simulink model "zad31"  (R2022b)
settings: Solver=FixedStepAuto  StartTime=0.0  StopTime=50  FixedStep=0.00001  RelTol=1e-3
model workspace (MAT data in the model file):
  a0 = 1
  a1 = 1
undefined symbols (not defined in the file): Ki, Kp
settings Model: Creator=vandm  LastModifiedBy=vandm

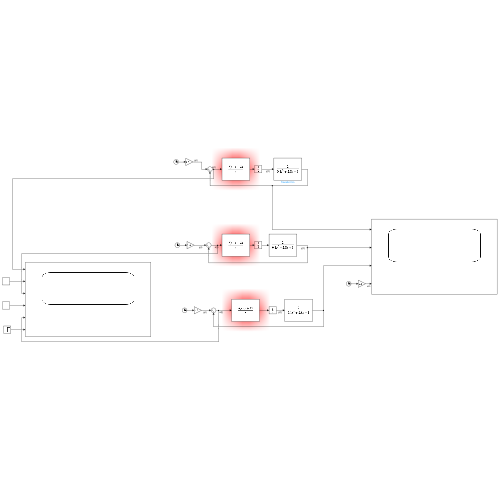
[thumbnail: Simulink's stored preview of the top-level diagram]
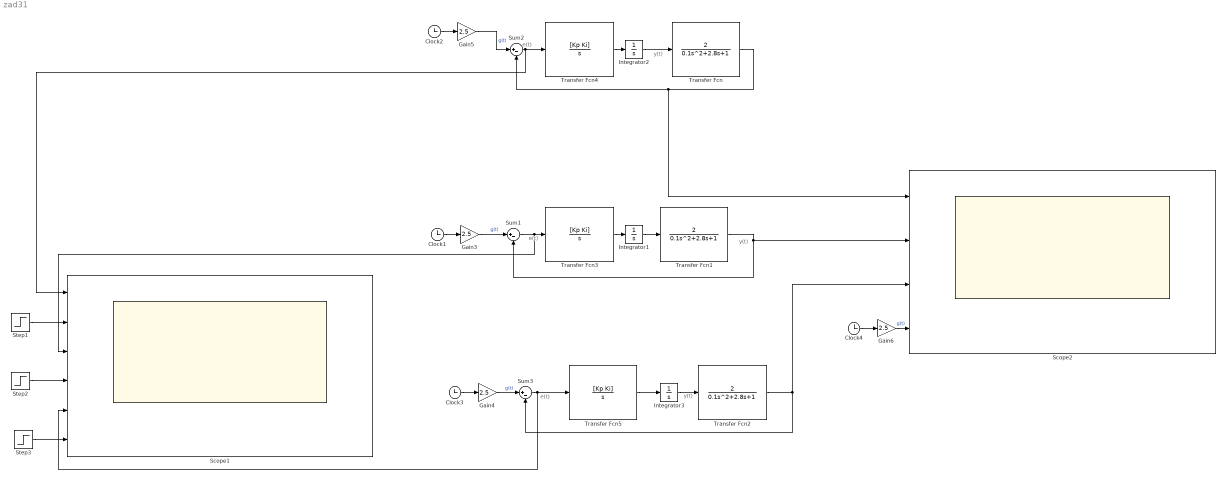
== system zad31 ==
  note: e(t)
  note: y(t)
  note: y(t)
  note: e(t)
  note: y(t)
  note: e(t)
  Clock{1..4} (4 alike) : Clock
  Gain{3..6} (4 alike) : Gain  Gain=2.5
  Integrator1 : Integrator
  Integrator2 : Integrator
  Integrator3 : Integrator
  Scope1 : Scope  NumInputPorts=6
  Scope2 : Scope  NumInputPorts=4
  Step1 : Step  Time=0  After=2.5/(2*1)  SampleTime=0
  Step2 : Step  Time=0  After=2.5/(2*5)  SampleTime=0
  Step3 : Step  Time=0  After=2.5/(2*10)  SampleTime=0
  Sum1 : Sum  Inputs=|+-
  Sum2 : Sum  Inputs=|+-
  Sum3 : Sum  Inputs=|+-
  Transfer Fcn : TransferFcn  Numerator=[2]  Denominator=[0.1 2.8 1]
  Transfer Fcn1 : TransferFcn  Numerator=[2]  Denominator=[0.1 2.8 1]
  Transfer Fcn2 : TransferFcn  Numerator=[2]  Denominator=[0.1 2.8 1]
  Transfer Fcn3 : TransferFcn  Numerator=[Kp Ki]  Denominator=[1 0]
  Transfer Fcn4 : TransferFcn  Numerator=[Kp Ki]  Denominator=[1 0]
  Transfer Fcn5 : TransferFcn  Numerator=[Kp Ki]  Denominator=[1 0]
  wires:
  Gain5/1 -> Sum2/1  "g(t)"
  Sum2/1 -> Transfer Fcn4/1, Scope1/1
  Integrator2/1 -> Transfer Fcn/1
  Transfer Fcn/1 -> Scope2/1, Sum2/2
  Gain3/1 -> Sum1/1  "g(t)"
  Integrator1/1 -> Transfer Fcn1/1
  Transfer Fcn1/1 -> Sum1/2, Scope2/2
  Transfer Fcn2/1 -> Sum3/2, Scope2/3
  Gain4/1 -> Sum3/1  "g(t)"
  Integrator3/1 -> Transfer Fcn2/1
  Sum3/1 -> Transfer Fcn5/1, Scope1/5
  Clock2/1 -> Gain5/1
  Clock1/1 -> Gain3/1
  Clock3/1 -> Gain4/1
  Step1/1 -> Scope1/2
  Step2/1 -> Scope1/4
  Step3/1 -> Scope1/6
  Clock4/1 -> Gain6/1
  Gain6/1 -> Scope2/4  "g(t)"
  Transfer Fcn4/1 -> Integrator2/1
  Transfer Fcn3/1 -> Integrator1/1
  Sum1/1 -> Transfer Fcn3/1, Scope1/3
  Transfer Fcn5/1 -> Integrator3/1
